simulink model "modele_chaine_base"  (R2024b)
settings: Solver=FixedStepDiscrete  StartTime=0.0  StopTime=(Nsim-1)*Tb  FixedStep=Te  RelTol=1e-3
values from neighbouring files (symbols this model uses):
  L = @(a, b) add_line(blk, a, b, 'autorouting', 'on')    [ajouter_codeur_registre.m]    (also in ajouter_decodeur_hamming.m; ajouter_modem_qpsk.m; ajouter_modem_qpsk_filtre.m; construire_modele_codeur_registre.m = @(a, b) add_line(mdl, a, b, 'autorouting', 'on'))
undefined symbols (not defined in the file or in its folder): A, dMid, dPhase, graine, sigma2e, Tb, Te
settings Model: Creator=youka  LastModifiedBy=youka

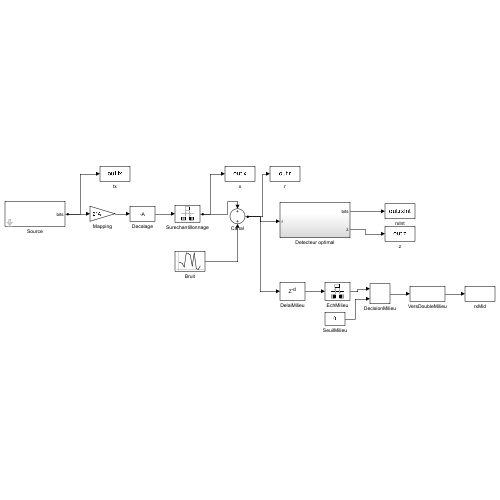
[thumbnail: Simulink's stored preview of the top-level diagram]
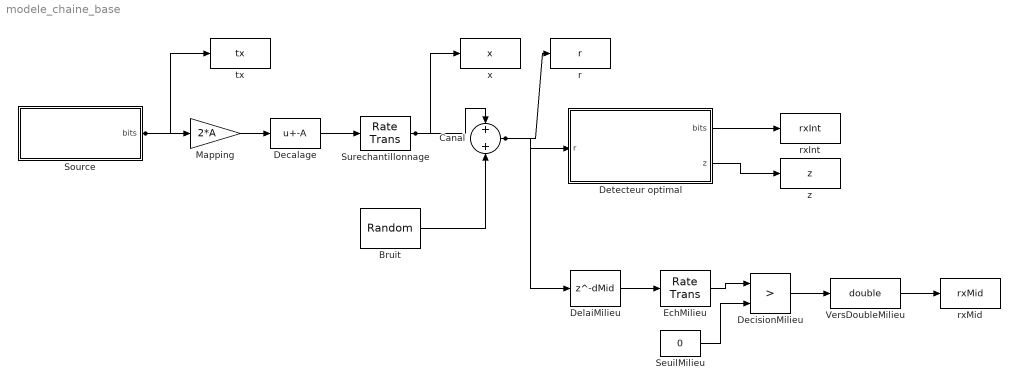
== system modele_chaine_base ==
  Bruit : RandomNumber  Variance=sigma2e  Seed=graine+1  SampleTime=Te
  Canal : Sum
  Decalage : Bias  Bias=-A  SaturateOnIntegerOverflow=off
  DecisionMilieu : RelationalOperator  Operator=>  OutDataTypeStr=boolean  RndMeth=Simplest  InputSameDT=off
  DelaiMilieu : Delay  DelayLength=dMid
  Detecteur optimal : Subsystem
  EchMilieu : RateTransition  OutPortSampleTime=Tb
  Mapping : Gain  Gain=2*A
  SeuilMilieu : Constant  Value=0  SampleTime=Tb
  Source : Subsystem  mask(Source binaire){p_m=0.5, Tb_m=Tb, graine_m=graine}
      mask prompts: p_m "Probabilité d'émettre un 1"; Tb_m "Durée d'un bit Tb (s)"; graine_m "Graine (Seed)"
      mask help: Source binaire sans mémoire : P(1) = p, un bit toutes les Tb secondes.
  Surechantillonnage : RateTransition  OutPortSampleTime=Te
  VersDoubleMilieu : DataTypeConversion  OutDataTypeStr=double  SaturateOnIntegerOverflow=off  RndMeth=Floor
  r : ToWorkspace  VariableName=r  SampleTime=-1
      settings: MaxDataPoints=20*L
  rxInt : ToWorkspace  VariableName=rxInt  SampleTime=-1
  rxMid : ToWorkspace  VariableName=rxMid  SampleTime=-1
  tx : ToWorkspace  VariableName=tx  SampleTime=-1
  x : ToWorkspace  VariableName=x  SampleTime=-1
      settings: MaxDataPoints=20*L
  z : ToWorkspace  VariableName=z  SampleTime=-1
  wires:
  Source/1(bits) -> tx/1, Mapping/1
  Mapping/1 -> Decalage/1
  Decalage/1 -> Surechantillonnage/1
  Surechantillonnage/1 -> Canal/1, x/1
  Bruit/1 -> Canal/2
  Canal/1 -> r/1, Detecteur optimal/1(r), DelaiMilieu/1
  Detecteur optimal/1(bits) -> rxInt/1
  Detecteur optimal/2(z) -> z/1
  DelaiMilieu/1 -> EchMilieu/1
  EchMilieu/1 -> DecisionMilieu/1
  SeuilMilieu/1 -> DecisionMilieu/2
  DecisionMilieu/1 -> VersDoubleMilieu/1
  VersDoubleMilieu/1 -> rxMid/1

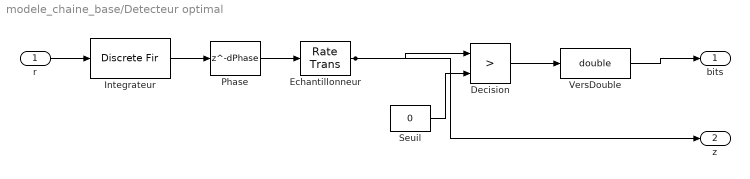
== system modele_chaine_base/Detecteur optimal ==
  r : Inport
  Decision : RelationalOperator  Operator=>  OutDataTypeStr=boolean  RndMeth=Simplest  InputSameDT=off
  Echantillonneur : RateTransition  OutPortSampleTime=Tb
  Integrateur : DiscreteFir  Coefficients=ones(1,L)/L
  Phase : Delay  DelayLength=dPhase
  Seuil : Constant  Value=0  SampleTime=Tb
  VersDouble : DataTypeConversion  OutDataTypeStr=double  SaturateOnIntegerOverflow=off  RndMeth=Floor
  bits : Outport
  z : Outport  Port=2
  wires:
  r/1 -> Integrateur/1
  Integrateur/1 -> Phase/1
  Phase/1 -> Echantillonneur/1
  Echantillonneur/1 -> Decision/1, z/1
  Seuil/1 -> Decision/2
  Decision/1 -> VersDouble/1
  VersDouble/1 -> bits/1

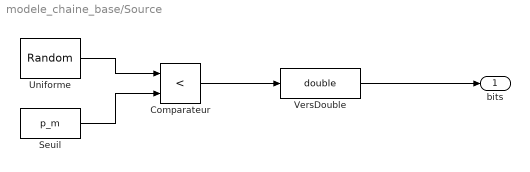
== system modele_chaine_base/Source ==
  Comparateur : RelationalOperator  Operator=<  OutDataTypeStr=boolean  RndMeth=Simplest  InputSameDT=off
  Seuil : Constant  Value=p_m  SampleTime=Tb_m
  Uniforme : UniformRandomNumber  Minimum=0  Seed=graine_m  SampleTime=Tb_m
  VersDouble : DataTypeConversion  OutDataTypeStr=double  SaturateOnIntegerOverflow=off  RndMeth=Floor
  bits : Outport
  wires:
  Uniforme/1 -> Comparateur/1
  Seuil/1 -> Comparateur/2
  Comparateur/1 -> VersDouble/1
  VersDouble/1 -> bits/1
